simulink subsystem "Spline_Path_Following_sub"  (R2023b)
settings: Solver=VariableStepAuto  StartTime=0.0  StopTime=10.0  RelTol=1e-3
undefined symbols (not defined in the file): Spline_Capture_Radius, Spline_Lookahead_Dist, Spline_Velocity_Axis
settings Model: Creator=ander  LastModifiedBy=ander

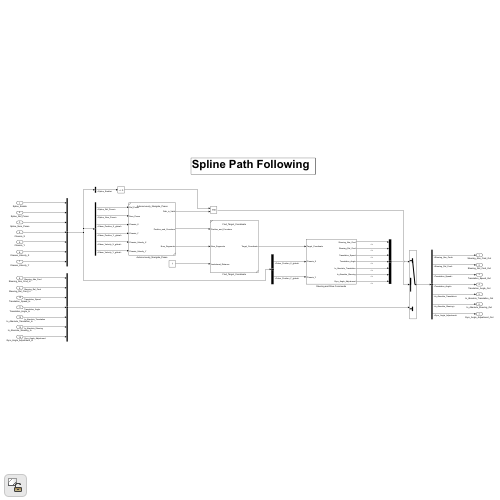
[thumbnail: Simulink's stored preview of the top-level diagram]
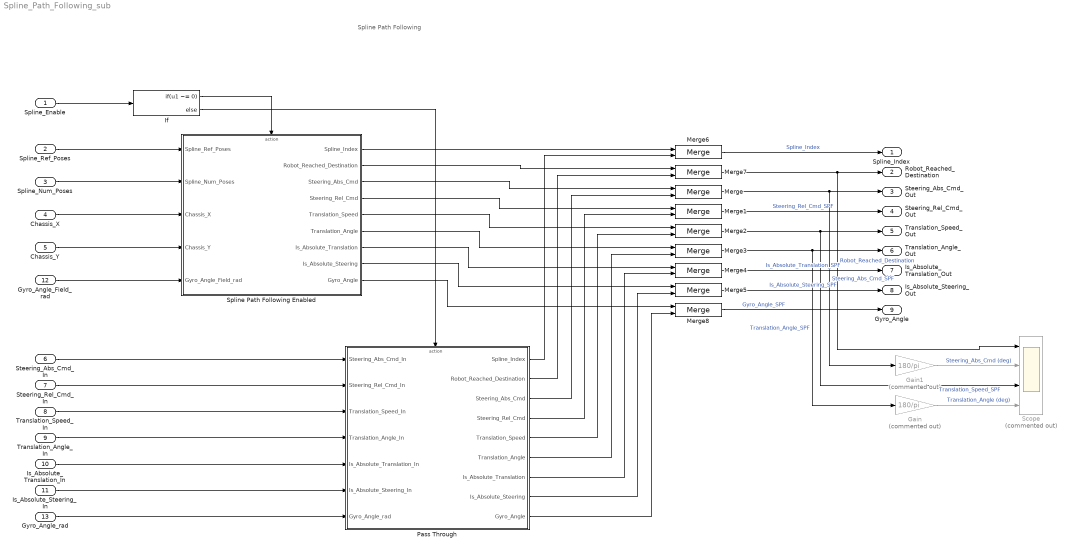
== system Spline_Path_Following_sub ==
  note: Spline Path Following
  Spline_Enable : Inport
  Spline_Ref_Poses : Inport  Port=2
  Spline_Num_Poses : Inport  Port=3
  Chassis_X : Inport  Port=4
  Chassis_Y : Inport  Port=5
  Steering_Abs_Cmd_In : Inport  Port=6
  Steering_Rel_Cmd_In : Inport  Port=7
  Translation_Speed_In : Inport  Port=8
  Translation_Angle_In : Inport  Port=9
  Is_Absolute_Translation_In : Inport  Port=10
  Is_Absolute_Steering_In : Inport  Port=11
  Gyro_Angle_Field_rad : Inport  Port=12
  Gyro_Angle_rad : Inport  Port=13
  Gain : Gain  Commented=on  Gain=180/pi
  Gain1 : Gain  Commented=on  Gain=180/pi
  If : If  IfExpression=u1 ~= 0
  Merge{,1..8} (9 alike) : Merge
  Pass Through : Subsystem
  Scope : Scope  Commented=on  NumInputPorts=4
  Spline Path Following Enabled : Subsystem
  Spline_Index : Outport
  Robot_Reached_Destination : Outport  Port=2
  Steering_Abs_Cmd_Out : Outport  Port=3
  Steering_Rel_Cmd_Out : Outport  Port=4
  Translation_Speed_Out : Outport  Port=5
  Translation_Angle_Out : Outport  Port=6
  Is_Absolute_Translation_Out : Outport  Port=7
  Is_Absolute_Steering_Out : Outport  Port=8
  Gyro_Angle : Outport  Port=9
  wires:
  Merge/1 -> Steering_Abs_Cmd_Out/1, Gain1/1  "Steering_Abs_Cmd_SPF"
  If/1 -> Spline Path Following Enabled/Action
  If/2 -> Pass Through/Action
  Steering_Abs_Cmd_In/1 -> Pass Through/1(Steering_Abs_Cmd_In)
  Steering_Rel_Cmd_In/1 -> Pass Through/2(Steering_Rel_Cmd_In)
  Translation_Speed_In/1 -> Pass Through/3(Translation_Speed_In)
  Translation_Angle_In/1 -> Pass Through/4(Translation_Angle_In)
  Is_Absolute_Translation_In/1 -> Pass Through/5(Is_Absolute_Translation_In)
  Is_Absolute_Steering_In/1 -> Pass Through/6(Is_Absolute_Steering_In)
  Spline Path Following Enabled/3(Steering_Abs_Cmd) -> Merge/1
  Pass Through/3(Steering_Abs_Cmd) -> Merge/2
  Spline Path Following Enabled/4(Steering_Rel_Cmd) -> Merge1/1
  Spline Path Following Enabled/5(Translation_Speed) -> Merge2/1
  Pass Through/4(Steering_Rel_Cmd) -> Merge1/2
  Spline Path Following Enabled/6(Translation_Angle) -> Merge3/1
  Pass Through/5(Translation_Speed) -> Merge2/2
  Pass Through/6(Translation_Angle) -> Merge3/2
  Spline Path Following Enabled/7(Is_Absolute_Translation) -> Merge4/1
  Pass Through/7(Is_Absolute_Translation) -> Merge4/2
  Spline Path Following Enabled/8(Is_Absolute_Steering) -> Merge5/1
  Pass Through/8(Is_Absolute_Steering) -> Merge5/2
  Merge1/1 -> Steering_Rel_Cmd_Out/1  "Steering_Rel_Cmd_SPF"
  Merge2/1 -> Translation_Speed_Out/1, Scope/3  "Translation_Speed_SPF"
  Merge3/1 -> Translation_Angle_Out/1, Gain/1  "Translation_Angle_SPF"
  Merge4/1 -> Is_Absolute_Translation_Out/1  "Is_Absolute_Translation_SPF"
  Merge5/1 -> Is_Absolute_Steering_Out/1  "Is_Absolute_Steering_SPF"
  Spline_Enable/1 -> If/1
  Spline_Ref_Poses/1 -> Spline Path Following Enabled/1(Spline_Ref_Poses)
  Spline_Num_Poses/1 -> Spline Path Following Enabled/2(Spline_Num_Poses)
  Chassis_X/1 -> Spline Path Following Enabled/3(Chassis_X)
  Chassis_Y/1 -> Spline Path Following Enabled/4(Chassis_Y)
  Spline Path Following Enabled/2(Robot_Reached_Destination) -> Merge7/1
  Pass Through/2(Robot_Reached_Destination) -> Merge7/2
  Merge7/1 -> Scope/1, Robot_Reached_Destination/1  "Robot_Reached_Destination"
  Gain/1 -> Scope/4  "Translation_Angle (deg)"
  Gain1/1 -> Scope/2  "Steering_Abs_Cmd (deg)"
  Gyro_Angle_rad/1 -> Pass Through/7(Gyro_Angle_rad)
  Gyro_Angle_Field_rad/1 -> Spline Path Following Enabled/5(Gyro_Angle_Field_rad)
  Spline Path Following Enabled/9(Gyro_Angle) -> Merge8/1
  Pass Through/9(Gyro_Angle) -> Merge8/2
  Merge8/1 -> Gyro_Angle/1  "Gyro_Angle_SPF"
  Merge6/1 -> Spline_Index/1  "Spline_Index"
  Spline Path Following Enabled/1(Spline_Index) -> Merge6/1
  Pass Through/1(Spline_Index) -> Merge6/2

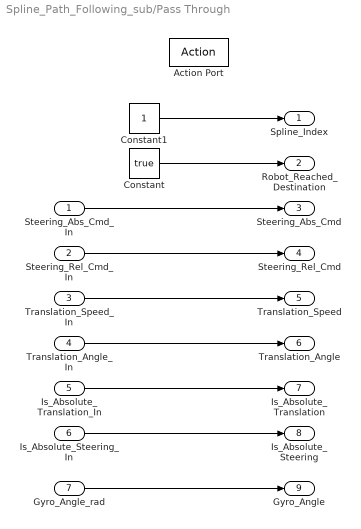
== system Spline_Path_Following_sub/Pass Through ==
  Steering_Abs_Cmd_In : Inport
  Steering_Rel_Cmd_In : Inport  Port=2
  Translation_Speed_In : Inport  Port=3
  Translation_Angle_In : Inport  Port=4
  Is_Absolute_Translation_In : Inport  Port=5
  Is_Absolute_Steering_In : Inport  Port=6
  Gyro_Angle_rad : Inport  Port=7
  Action Port : ActionPort
  Constant : Constant  Value=true
  Constant1 : Constant
  Spline_Index : Outport
  Robot_Reached_Destination : Outport  Port=2
  Steering_Abs_Cmd : Outport  Port=3
  Steering_Rel_Cmd : Outport  Port=4
  Translation_Speed : Outport  Port=5
  Translation_Angle : Outport  Port=6
  Is_Absolute_Translation : Outport  Port=7
  Is_Absolute_Steering : Outport  Port=8
  Gyro_Angle : Outport  Port=9
  wires:
  Constant1/1 -> Spline_Index/1
  Gyro_Angle_rad/1 -> Gyro_Angle/1
  Constant/1 -> Robot_Reached_Destination/1
  Is_Absolute_Steering_In/1 -> Is_Absolute_Steering/1
  Is_Absolute_Translation_In/1 -> Is_Absolute_Translation/1
  Translation_Angle_In/1 -> Translation_Angle/1
  Translation_Speed_In/1 -> Translation_Speed/1
  Steering_Rel_Cmd_In/1 -> Steering_Rel_Cmd/1
  Steering_Abs_Cmd_In/1 -> Steering_Abs_Cmd/1

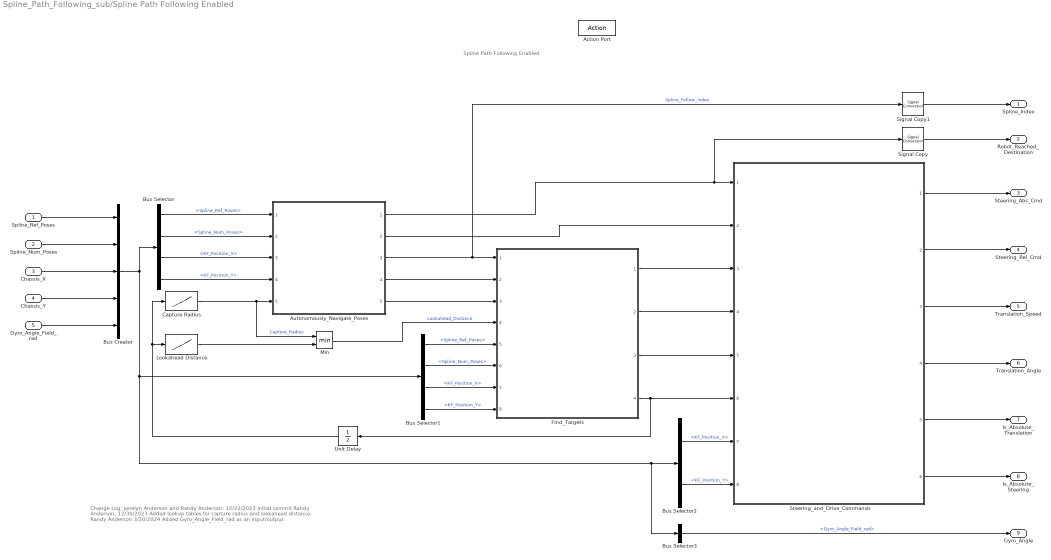
== system Spline_Path_Following_sub/Spline Path Following Enabled ==
  note: Change Log:
      | Janelyn Anderson and Randy Anderson: 12/23/2023
      | Initial commit
      | Randy Anderson, 12/30/2023
      | Added lookup tables for capture radius and lookahead distance.
      | Randy Anderson 3/20/2024
      | Added Gyro_Angle_Field_rad as an input/output
  note: Spline Path Following Enabled
  Spline_Ref_Poses : Inport
  Spline_Num_Poses : Inport  Port=2
  Chassis_X : Inport  Port=3
  Chassis_Y : Inport  Port=4
  Gyro_Angle_Field_rad : Inport  Port=5
  Action Port : ActionPort  InitializeStates=reset  PropagateVarSize=During execution
  Autonomously_Navigate_Poses : Subsystem  ReferencedSubsystem=Autonomously_Navigate_Poses
  Bus Creator : BusCreator  Inputs=5
  Bus Selector : BusSelector  OutputSignals=Spline_Ref_Poses,Spline_Num_Poses,KF_Position_X,KF_Position_Y
  Bus Selector1 : BusSelector  OutputSignals=Spline_Ref_Poses,Spline_Num_Poses,KF_Position_X,KF_Position_Y
  Bus Selector2 : BusSelector  OutputSignals=KF_Position_X,KF_Position_Y
  Bus Selector3 : BusSelector  OutputSignals=Gyro_Angle_Field_rad
  Capture Radius : Lookup_n-D  NumberOfTableDimensions=1  BreakpointsForDimension1=Spline_Velocity_Axis  Table=Spline_Capture_Radius  ExtrapMethod=Clip  InternalRulePriority=Speed  RndMeth=Simplest
  Find_Targets : Subsystem  ReferencedSubsystem=Find_Target_Position_Velocity_Heading
  Lookahead Distance : Lookup_n-D  NumberOfTableDimensions=1  BreakpointsForDimension1=Spline_Velocity_Axis  Table=Spline_Lookahead_Dist  ExtrapMethod=Clip  InternalRulePriority=Speed  RndMeth=Simplest
  Min : MinMax  Inputs=2
  Signal Copy : SignalConversion  OverrideOpt=off
  Signal Copy1 : SignalConversion  OverrideOpt=off
  Steering_and_Drive_Commands : Subsystem  ReferencedSubsystem=Spline_Steering_and_Drive_Commands
  Unit Delay : UnitDelay  SampleTime=-1  HasFrameUpgradeWarning=on
  Spline_Index : Outport
  Robot_Reached_Destination : Outport  Port=2
  Steering_Abs_Cmd : Outport  Port=3
  Steering_Rel_Cmd : Outport  Port=4
  Translation_Speed : Outport  Port=5
  Translation_Angle : Outport  Port=6
  Is_Absolute_Translation : Outport  Port=7
  Is_Absolute_Steering : Outport  Port=8
  Gyro_Angle : Outport  Port=9
  wires:
  Signal Copy1/1 -> Spline_Index/1
  Bus Selector3/1 -> Gyro_Angle/1  "<Gyro_Angle_Field_rad>"
  Gyro_Angle_Field_rad/1 -> Bus Creator/5
  Min/1 -> Find_Targets/4  "Lookahead_Distance"
  Lookahead Distance/1 -> Min/2
  Unit Delay/1 -> Capture Radius/1, Lookahead Distance/1
  Capture Radius/1 -> Min/1, Autonomously_Navigate_Poses/5  "Capture_Radius"
  Bus Selector2/2 -> Steering_and_Drive_Commands/8  "<KF_Position_Y>"
  Bus Selector2/1 -> Steering_and_Drive_Commands/7  "<KF_Position_X>"
  Bus Selector1/4 -> Find_Targets/8  "<KF_Position_Y>"
  Bus Selector1/3 -> Find_Targets/7  "<KF_Position_X>"
  Bus Selector/4 -> Autonomously_Navigate_Poses/4  "<KF_Position_Y>"
  Bus Selector/3 -> Autonomously_Navigate_Poses/3  "<KF_Position_X>"
  Autonomously_Navigate_Poses/2 -> Steering_and_Drive_Commands/2
  Signal Copy/1 -> Robot_Reached_Destination/1
  Bus Selector1/1 -> Find_Targets/5  "<Spline_Ref_Poses>"
  Bus Selector1/2 -> Find_Targets/6  "<Spline_Num_Poses>"
  Bus Selector/1 -> Autonomously_Navigate_Poses/1  "<Spline_Ref_Poses>"
  Bus Selector/2 -> Autonomously_Navigate_Poses/2  "<Spline_Num_Poses>"
  Bus Creator/1 -> Bus Selector1/1, Bus Selector2/1, Bus Selector3/1, Bus Selector/1
  Chassis_Y/1 -> Bus Creator/4
  Chassis_X/1 -> Bus Creator/3
  Spline_Num_Poses/1 -> Bus Creator/2
  Spline_Ref_Poses/1 -> Bus Creator/1
  Find_Targets/3 -> Steering_and_Drive_Commands/5
  Find_Targets/4 -> Steering_and_Drive_Commands/6, Unit Delay/1
  Autonomously_Navigate_Poses/3 -> Find_Targets/1, Signal Copy1/1  "Spline_Follow_Index"
  Autonomously_Navigate_Poses/1 -> Steering_and_Drive_Commands/1, Signal Copy/1
  Steering_and_Drive_Commands/4 -> Translation_Angle/1
  Steering_and_Drive_Commands/1 -> Steering_Abs_Cmd/1
  Steering_and_Drive_Commands/3 -> Translation_Speed/1
  Steering_and_Drive_Commands/6 -> Is_Absolute_Steering/1
  Steering_and_Drive_Commands/2 -> Steering_Rel_Cmd/1
  Find_Targets/2 -> Steering_and_Drive_Commands/4
  Autonomously_Navigate_Poses/4 -> Find_Targets/2
  Steering_and_Drive_Commands/5 -> Is_Absolute_Translation/1
  Find_Targets/1 -> Steering_and_Drive_Commands/3
  Autonomously_Navigate_Poses/5 -> Find_Targets/3
